simulink model "Bike2DOF_s"  (R2023a)
settings: Solver=VariableStepAuto  StartTime=0.0  StopTime=10.0  RelTol=1e-3
undefined symbols (not defined in the file): Iz, l_f, l_r, m
settings Model: Creator=Tan_Tram  LastModifiedBy=Tan_Tram

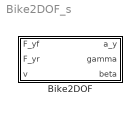
== system Bike2DOF_s ==
  Bike2DOF : Subsystem

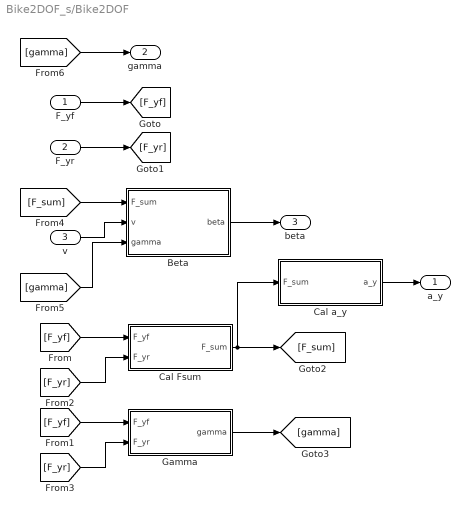
== system Bike2DOF_s/Bike2DOF ==
  F_yf : Inport
  F_yr : Inport  Port=2
  v : Inport  Port=3
  Beta : Subsystem
  Cal Fsum : Subsystem
  Cal a_y : Subsystem
  Gamma : Subsystem
  a_y : Outport
  gamma : Outport  Port=2
  beta : Outport  Port=3
  wires:
  F_yr/1 -> [F_yr]
  [F_yf] -> Cal Fsum/1(F_yf)
  [F_sum] -> Beta/1(F_sum)
  [gamma] -> gamma/1
  F_yf/1 -> [F_yf]
  v/1 -> Beta/2(v)
  [F_yr] -> Cal Fsum/2(F_yr)
  [gamma] -> Beta/3(gamma)
  [F_yf] -> Gamma/1(F_yf)
  [F_yr] -> Gamma/2(F_yr)
  Beta/1(beta) -> beta/1
  Cal Fsum/1(F_sum) -> Cal a_y/1(F_sum), [F_sum]
  Gamma/1(gamma) -> [gamma]
  Cal a_y/1(a_y) -> a_y/1

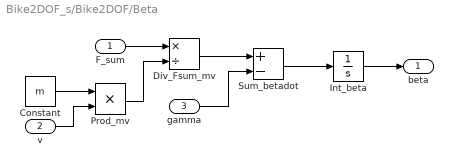
== system Bike2DOF_s/Bike2DOF/Beta ==
  F_sum : Inport
  v : Inport  Port=2
  gamma : Inport  Port=3
  Constant : Constant  Value=m
  Div_Fsum_mv : Product  Inputs=*/
  Int_beta : Integrator
  Prod_mv : Product  Inputs=**
  Sum_betadot : Sum  Inputs=+-
  beta : Outport
  wires:
  Sum_betadot/1 -> Int_beta/1
  Constant/1 -> Prod_mv/1
  Int_beta/1 -> beta/1
  v/1 -> Prod_mv/2
  Div_Fsum_mv/1 -> Sum_betadot/1
  F_sum/1 -> Div_Fsum_mv/1
  Prod_mv/1 -> Div_Fsum_mv/2
  gamma/1 -> Sum_betadot/2

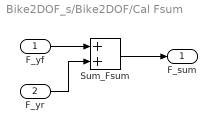
== system Bike2DOF_s/Bike2DOF/Cal Fsum ==
  F_yf : Inport
  F_yr : Inport  Port=2
  Sum_Fsum : Sum
  F_sum : Outport
  wires:
  F_yr/1 -> Sum_Fsum/2
  F_yf/1 -> Sum_Fsum/1
  Sum_Fsum/1 -> F_sum/1

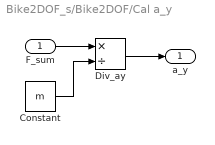
== system Bike2DOF_s/Bike2DOF/Cal a_y ==
  F_sum : Inport
  Constant : Constant  Value=m
  Div_ay : Product  Inputs=*/
  a_y : Outport
  wires:
  Div_ay/1 -> a_y/1
  Constant/1 -> Div_ay/2
  F_sum/1 -> Div_ay/1

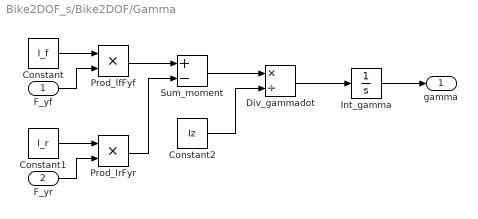
== system Bike2DOF_s/Bike2DOF/Gamma ==
  F_yf : Inport
  F_yr : Inport  Port=2
  Constant : Constant  Value=l_f
  Constant1 : Constant  Value=l_r
  Constant2 : Constant  Value=Iz
  Div_gammadot : Product  Inputs=*/
  Int_gamma : Integrator
  Prod_lfFyf : Product  Inputs=**
  Prod_lrFyr : Product  Inputs=**
  Sum_moment : Sum  Inputs=+-
  gamma : Outport
  wires:
  Prod_lfFyf/1 -> Sum_moment/1
  F_yf/1 -> Prod_lfFyf/2
  Constant/1 -> Prod_lfFyf/1
  Int_gamma/1 -> gamma/1
  Constant1/1 -> Prod_lrFyr/1
  F_yr/1 -> Prod_lrFyr/2
  Constant2/1 -> Div_gammadot/2
  Prod_lrFyr/1 -> Sum_moment/2
  Sum_moment/1 -> Div_gammadot/1
  Div_gammadot/1 -> Int_gamma/1
